simulink model "bldc_current_control"  (R2026a)
settings: Solver=FixedStepDiscrete  StopTime=5  FixedStep=Ts_sim
InitFcn:
  | warning('off','physmod:simscape:engine:core:advancer_errors:fallback_solve')
model workspace (MAT data in the model file):
  B_rotor = 2e-07
  B_turntable = 5e-06
  C_buck = 4.7e-05
  Dmax = 0.95
  Fsw = 50000
  I_max = 1.5
  J_body = 0.002
  J_flywheel = 0.00012
  J_rotor = 5e-07
  K_A = 1
  Ki_current = 7539.82236862
  Ki_speed = 4.0575
  Kp_current = 0.753982236862
  Kp_speed = 0.111675
  L_buck = 0.0001
  T_brk_turntable = 0.0012
  T_col_turntable = 0.001
  Ts_inner = 1e-05
  Ts_outer = 0.01
  Ts_sim = 2e-06
  Vin = 12
  f_pwm = 5000
  psi_m = 0.004
  slew_acc_max = 1.2
  slew_rate_max = 0.5
  w_bias = 0
  w_max = 600
libraries: nesl_utility x18, fl_lib x17, ee_lib x13, slpidlib x3, simulink x1, eePwmGenerator x1
(part 1 of 2)
settings Model: Creator=mulusoy  LastModifiedBy=tama
settings SimscapeCC: SimscapeNominalValues="[{\"value\":\"1\",\"unit\":\"A\"},{\"value\":\"1\",\"unit\":\"bar\"},{\"value\":\"1\",\"unit\":\"cm^2\"},{\"value\":\"1\",\"unit\":\"cm^3/s\"},{\"value\":\"1\",\"unit\":\"kJ/kg\"},{\"value\":\"1\",\"unit\":\"kW\"},{\"value\":\"1\",\"unit\":\"l\"},{\"value\":\"1\",\"unit\":\"N\"},{\"value\":\"1\",\"unit\":\"N*m\"},{\"value\":\"1\",\"unit\":\"V\"}]"  SimscapeLogType=none  SimscapeLogDataHistory=5000.0

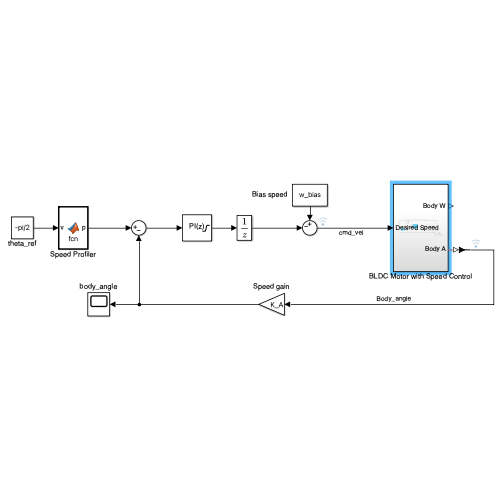
[thumbnail: Simulink's stored preview of the top-level diagram]
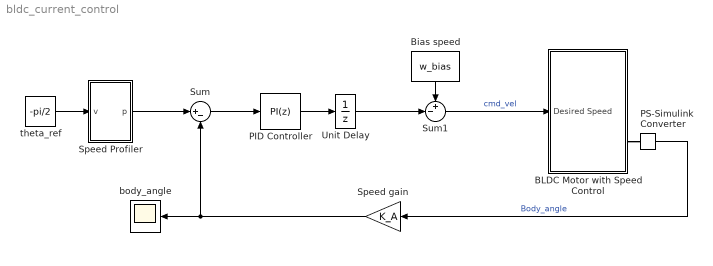
== system bldc_current_control ==
  BLDC Motor with Speed Control : Subsystem
  Bias speed : Constant  Value=w_bias
  PID Controller : slpidlib/PID Controller  Controller=PI  Form=Parallel  TimeDomain=Discrete-time  UseExternalTs=off  SampleTime=0.01  IntegratorMethod=Forward Euler  FilterMethod=Forward Euler  ControllerParametersSource=internal  P=2861  I=6984  UseKiTs=off  D=0  UseExternalDerivativeSource=off  N=100  UseFilter=on  TunerSelectOption=Transfer Function Based (PID Tuner App)  InitialConditionSource=internal  InitialConditionForIntegrator=0  InitialConditionForFilter=0  DifferentiatorICPrevScaledInput=0  ExternalReset=none  TrackingMode=off  Kt=1  LimitOutput=on  SatLimitsSource=internal  UpperSaturationLimit=w_max  LowerSaturationLimit=-w_max  LinearizeAsGain=on  AntiWindupMode=clamping  Kb=1  LimitIntegrator=off  UpperIntegratorSaturationLimit=inf  LowerIntegratorSaturationLimit=-inf  POutMin=[]  POutMax=[]  IOutMin=[]  IOutMax=[]  DOutMin=[]  DOutMax=[]  NOutMin=[]  NOutMax=[]  SumOutMin=[]  SumOutMax=[]  SaturationOutMin=[]  SaturationOutMax=[]  PParamMin=[]  PParamMax=[]  IParamMin=[]  IParamMax=[]  DParamMin=[]  DParamMax=[]  NParamMin=[]  NParamMax=[]  KbParamMin=[]  KbParamMax=[]  KtParamMin=[]  KtParamMax=[]  KbOutMin=[]  KbOutMax=[]  KtOutMin=[]  KtOutMax=[]  IntegratorOutMin=[]  IntegratorOutMax=[]  FilterOutMin=[]  FilterOutMax=[]  SumI1OutMin=[]  SumI1OutMax=[]  SumI2OutMin=[]  SumI2OutMax=[]  SumI3OutMin=[]  SumI3OutMax=[]  SumI4OutMin=[]  SumI4OutMax=[]  SumDOutMin=[]  SumDOutMax=[]  DifferentiatorOutMin=[]  DifferentiatorOutMax=[]  FilterDiffOutCoefMin=[]  FilterDiffOutCoefMax=[]  ReciprocalOutMin=[]  ReciprocalOutMax=[]  SumDenOutMin=[]  SumDenOutMax=[]  SumNumOutMin=[]  SumNumOutMax=[]  DivideOutMin=[]  DivideOutMax=[]  UdiffTsProdOutMin=[]  UdiffTsProdOutMax=[]  NTsProdOutMin=[]  NTsProdOutMax=[]  UintegralTsProdOutMin=[]  UintegralTsProdOutMax=[]  UngainTsProdOutMin=[]  UngainTsProdOutMax=[]  ClampingZeroOutDataTypeStr=Inherit: Inherit via back propagation  ClampingZeroOutMin=[]  ClampingZeroOutMax=[]  FilterDenConstantOutDataTypeStr=Inherit: Inherit via back propagation  FilterDenConstantOutMin=[]  FilterDenConstantOutMax=[]  PCopyOutDataTypeStr=Inherit: Inherit via back propagation  PCopyOutMin=[]  PCopyOutMax=[]  NCopyOutDataTypeStr=Inherit: Inherit via back propagation  NCopyOutMin=[]  NCopyOutMax=[]  IntegratorContinuousStateAttributes=''  IntegratorStateMustResolveToSignalObject=off  IntegratorRTWStateStorageClass=Auto  FilterContinuousStateAttributes=''  FilterStateMustResolveToSignalObject=off  FilterRTWStateStorageClass=Auto  ParallelPVariant=InternalParameters  IdealPVariant=Disabled  IVariant=InternalParameters  DVariant=Disabled  IntegratorVariant=Discrete  SatVariant=Enabled  AWVariant=DiscClampingParallel  PCopyVariant=Disabled  TRVariant=Disabled  FdbkBlocksVariant=Forward  IdealPFdbkVariant=Disabled  SatFdbkVariant=Disabled  DerivativeFilterVariant=Disabled  NVariant=Disabled  NCopyVariant=Disabled_SignalSpec  FilterICVariant=Disabled  IntegratorICVariant=InternalICs  ExternalResetVariant=Disabled  TRSumVariant=Passthrough  SumFdbkVariant=Disabled  SumVariant=Sum_PI  TsampFilterVariant=InternalTs  TsampNgainVariant=Passthrough  TsampIntegralVariant=Disabled_SignalSpec  ExternalSaturationOutDataTypeStr=Inherit: Same as second input  DerivativeSourceVariant=Disabled  PreIntVariant=InternalPreInt
  PS-Simulink Converter : nesl_utility/PS-Simulink Converter  PhysicalDomain=network_engine_domain  SubClassName=ps_output  LeftPortType=input  RightPortType=output  PseudoPeriodic=off  Frequencies=[]  VectorFormat=inherit  Unit=inherit  AffineConversion=off
  Speed Profiler : MATLAB Function  TreatAsAtomicUnit=on  SystemSampleTime=Ts_outer
  Speed gain : Gain  Gain=K_A
  Sum : Sum  Inputs=|+-
  Sum1 : Sum  Inputs=+-|
  Unit Delay : UnitDelay  SampleTime=-1
  body_angle : Scope
      settings: ActiveDisplayYMinimum=-1.3977070447201263  ActiveDisplayYMaximum=0.52158832632188012  DataLoggingVariableName=ScopeData3
  theta_ref : Constant  Value=-pi/2
  wires:
  PID Controller/1 -> Unit Delay/1
  PS-Simulink Converter/1 -> Speed gain/1  "Body_angle"
  theta_ref/1 -> Speed Profiler/1(v)
  Sum/1 -> PID Controller/1
  Speed gain/1 -> Sum/2, body_angle/1
  Bias speed/1 -> Sum1/1
  Unit Delay/1 -> Sum1/2
  Sum1/1 -> BLDC Motor with Speed Control/1(Desired Speed)  "cmd_vel"
  Speed Profiler/1(p) -> Sum/1
  connections:
  BLDC Motor with Speed Control/RConn2 -- PS-Simulink Converter/LConn1

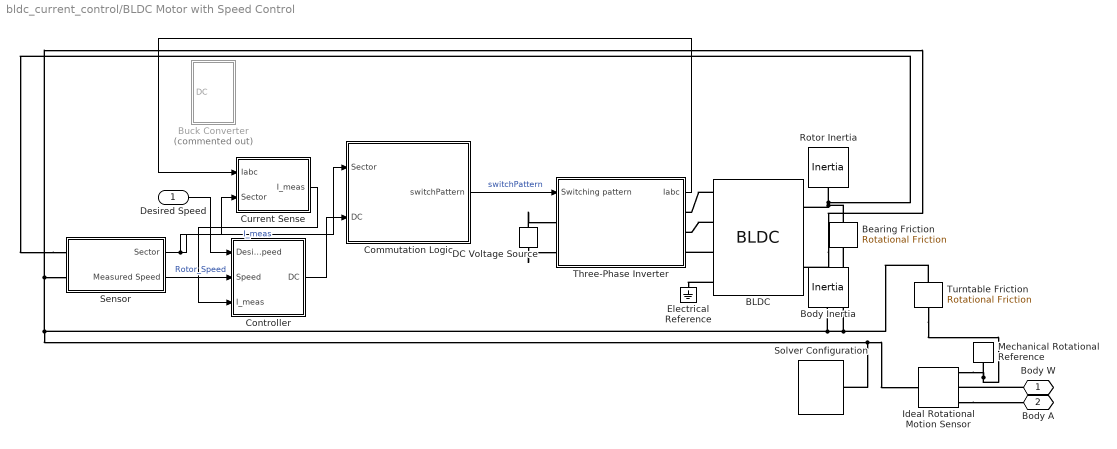
== system bldc_current_control/BLDC Motor with Speed Control ==
  Desired Speed : Inport
  BLDC : ee_lib/Electromechanical/Permanent Magnet/BLDC  port_option=ee.enum.threePhasePort.expanded  rotor_param=1  pm_flux_linkage=psi_m Wb  theta_constant=120/1 deg  emf_max=9.6 V  w_meas=600 rpm  DphiDtheta_tab=[0, -.1528, -.1528, .1528, .1528, 0] Wb/rad  back_emf_tab=[0, -9.6, -9.6, 9.6, 9.6, 0] V  rotor_angle_tab=[0, 7.5, 22.5, 37.5, 52.5, 60] deg  nPolePairs=1  axes_param=2  winding_type=ee.enum.statorconnection.wye  stator_param=ee.enum.statorparam.LdLqL0  machine_param=ee.enum.dqparameterization.constant  Ld=0.2 mH  Lq=0.2 mH  idVec=[-200, 0, 200] A  iqVec=[-200, 0, 200] A  LdMatrix=0.00022 * ones(3, 3) H  LqMatrix=0.00022 * ones(3, 3) H  L0=0.2 mH  Ls=0.0002 H  Lm=0 H  Ms=0.00002 H  Rs=2 Ohm  zero_sequence=ee.enum.park.zerosequence.include  loss_param=ee.enum.ironloss.none  losses_oc=[0, 0, 0] W  losses_sc=[0, 0, 0] W  f_losses=60 Hz  Isc_losses=95 A  J=0 kg*m^2  lam=B_rotor N*m/(rad/s)  i_d_specify=off  i_d_priority=None  i_d=0 A  i_d_nominal_specify=off  i_d_nominal_value=1  i_d_nominal_unit=A  i_q_specify=off  i_q_priority=None  i_q=0 A  i_q_nominal_specify=off  i_q_nominal_value=1  i_q_nominal_unit=A  torque_specify=off  torque_priority=None  torque=0 N*m  torque_nominal_specify=off  torque_nominal_value=1  torque_nominal_unit=N*m  angular_velocity_specify=on  angular_velocity_priority=High  angular_velocity=w_bias rpm  angular_velocity_nominal_specify=off  angular_velocity_nominal_value=1  angular_velocity_nominal_unit=rpm  angular_position_specify=off  angular_position_priority=High  angular_position=0 deg  angular_position_nominal_specify=off  angular_position_nominal_value=1  angular_position_nominal_unit=deg  alpha=3.93e-3 1/K  alpha_flux=-0.001 1/K  Tmeas=298.15 K  stator_thermal_mass=100 J/K  rotor_thermal_mass=200 J/K  Rm_percent_rotor=90  Rd_percent_rotor=30  temperatureA_specify=off  temperatureA_priority=High  temperatureA=25 degC  temperatureA_nominal_specify=off  temperatureA_nominal_value=1  temperatureA_nominal_unit=degC  temperatureB_specify=off  temperatureB_priority=High  temperatureB=25 degC  temperatureB_nominal_specify=off  temperatureB_nominal_value=1  temperatureB_nominal_unit=degC  temperatureC_specify=off  temperatureC_priority=High  temperatureC=25 degC  temperatureC_nominal_specify=off  temperatureC_nominal_value=1  temperatureC_nominal_unit=degC  temperatureR_specify=off  temperatureR_priority=High  temperatureR=25 degC  temperatureR_nominal_specify=off  temperatureR_nominal_value=1  temperatureR_nominal_unit=degC
  Bearing Friction : fl_lib/Mechanical/Rotational Elements/Rotational Friction  brkwy_trq=0.05 m*mN  brkwy_vel=0.1 rad/s  Col_trq=0.05 m*mN  visc_coef=0 N*m*s/rad  w_specify=off  w_priority=None  w=0 rad/s  w_nominal_specify=off  w_nominal_value=1  w_nominal_unit=rad/s  t_specify=off  t_priority=None  t=0 N*m  t_nominal_specify=off  t_nominal_value=1  t_nominal_unit=N*m
  Body Inertia : fl_lib/Mechanical/Rotational Elements/Inertia  inertia=J_body kg*m^2  num_ports=foundation.enum.numPorts2.one  w_specify=on  w_priority=High  w=0 rad/s  w_nominal_specify=off  w_nominal_value=1  w_nominal_unit=rad/s  t_specify=off  t_priority=None  t=0 N*m  t_nominal_specify=off  t_nominal_value=1  t_nominal_unit=N*m
  Buck Converter : Subsystem  Description=Label-mode variant. Averaged (default): Vin*d controlled source + L/C filter, run with Ts_sim = 1e-5. Switching: PWM + MOSFETs at Fsw, needs Ts_sim <= 2e-7 (1% duty resolution at 50 kHz) - set Ts_sim in the model workspace before switching.  Commented=on  Variant=on  VariantControlMode=label  LabelModeActiveChoice=Averaged
  Commutation Logic : Subsystem
  Controller : Subsystem
  Current Sense : Subsystem
  DC Voltage Source : ee_lib/Additional Components/SPICE Sources/DC Voltage Source  DC=Vin V
  Electrical Reference : fl_lib/Electrical/Electrical Elements/Electrical Reference
  Ideal Rotational Motion Sensor : fl_lib/Mechanical/Mechanical Sensors/Ideal Rotational Motion Sensor  reference=foundation.enum.MeasurementReference.difference  acceleration_port=false  velocity_port=true  position_port=true  wrap_angle=false  offset=0 rad
  Mechanical Rotational Reference : fl_lib/Mechanical/Rotational Elements/Mechanical Rotational Reference
  Rotor Inertia : fl_lib/Mechanical/Rotational Elements/Inertia  inertia=J_flywheel + J_rotor kg*m^2  num_ports=foundation.enum.numPorts2.one  w_specify=on  w_priority=High  w=w_bias rpm  w_nominal_specify=off  w_nominal_value=1  w_nominal_unit=rad/s  t_specify=off  t_priority=None  t=0 N*m  t_nominal_specify=off  t_nominal_value=1  t_nominal_unit=N*m
  Sensor : Subsystem
  Solver Configuration : nesl_utility/Solver Configuration  PhysicalDomain=network_engine_domain  SubClassName=solver  LeftPortType=input  RightPortType=generic  Tones=[]  Harmonics=[]  SimulateNoise=off  Profile=off  UseLocalSampling=off  EnableSwitchedLinearOptims=on  FrequencyDomain=off  UseCCode=off  RelTol=0.001  AbsTol=1e-06  MinStep=1e-09  ToWorkspace=off  RevertToSquareIcSolve=off  NumHomotopyIterations=100  PhasorMode=off  PhasorModeNumHarmonics=1  ConsistencySolver=NEWTON_FTOL  CanonicalOrdering=UNORDERED  OptimizeIntermediates=UNOPTIMIZED  IndexReductionMethod=DerivativeReplacement  DoDC=off  ResidualTolerance=1e-09  ConsistencyTolSource=GLOBAL  ConsistencyAbsTol=0.001  ConsistencyRelTol=0.001  ConsistencyTolFactor=0.001  UseLocalSolver=on  LocalSolverChoice=NE_BACKWARD_EULER_ADVANCER  ResolveIndetEquations=on  FunctionEvalNumThread=1  LocalSolverSampleTime=Ts_sim  DoFixedCost=on  MaxNonlinIter=4  MaxModeIter=2  ComputeImpulses=off  ImpulseIterations=2  LinearAlgebra=auto  LinearAlgebraNumThread=0  EquationFormulation=NE_TIME_EF  DelaysMemoryBudget=1024  AutomaticFiltering=off  FilteringTimeConstant=0.001  PartitionStorageMethod=AS_NEEDED  PartitionMemoryBudget=1024  PartitionMethod=ROBUST  MultibodyUseLocalSolver=off  MultibodyLocalSolverChoice=ODE1  MultibodyLocalSolverSampleTime=0.001
  Three-Phase Inverter : Subsystem
  Turntable Friction : fl_lib/Mechanical/Rotational Elements/Rotational Friction  brkwy_trq=T_brk_turntable N*m  brkwy_vel=0.1 rad/s  Col_trq=T_col_turntable N*m  visc_coef=B_turntable N*m*s/rad  w_specify=off  w_priority=None  w=0 rad/s  w_nominal_specify=off  w_nominal_value=1  w_nominal_unit=rad/s  t_specify=off  t_priority=None  t=0 N*m  t_nominal_specify=off  t_nominal_value=1  t_nominal_unit=N*m
  Body W : PMIOPort  Side=Right
  Body A : PMIOPort  Port=2  Side=Right
  wires:
  Commutation Logic/1(switchPattern) -> Three-Phase Inverter/1(Switching pattern)  "switchPattern"
  Current Sense/1(I_meas) -> Controller/3(I_meas)  "I_meas"
  Three-Phase Inverter/1(Iabc) -> Current Sense/1(Iabc)
  Desired Speed/1 -> Controller/1(Desired Speed)
  Controller/1(DC) -> Commutation Logic/2(DC)
  Sensor/1(Sector) -> Current Sense/2(Sector), Commutation Logic/1(Sector)
  Sensor/2(Measured Speed) -> Controller/2(Speed)  "Rotor_Speed"
  connections:
  BLDC/LConn2 -- Three-Phase Inverter/RConn2
  BLDC/LConn1 -- Three-Phase Inverter/RConn1
  BLDC/LConn4 -- Electrical Reference/LConn1
  BLDC/LConn3 -- Three-Phase Inverter/RConn3
  Mechanical Rotational Reference/LConn1 -- Ideal Rotational Motion Sensor/RConn1 -- Turntable Friction/RConn1
  Body W/RConn1 -- Ideal Rotational Motion Sensor/RConn2
  Ideal Rotational Motion Sensor/RConn3 -- Body A/RConn1
  DC Voltage Source/LConn1 -- Three-Phase Inverter/LConn1
  DC Voltage Source/RConn1 -- Three-Phase Inverter/LConn2
  Sensor/LConn1 -- Bearing Friction/LConn1 -- BLDC/RConn1 -- Rotor Inertia/LConn1
  Body Inertia/LConn1 -- Ideal Rotational Motion Sensor/LConn1 -- Solver Configuration/RConn1 -- Turntable Friction/LConn1 -- Bearing Friction/RConn1 -- BLDC/RConn2 -- Sensor/LConn2

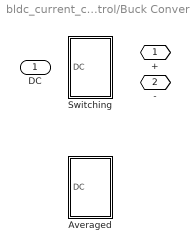
== system bldc_current_control/BLDC Motor with Speed Control/Buck Converter ==
  DC : Inport
  Averaged : Subsystem  VariantControl=Averaged
  Switching : Subsystem  VariantControl=Switching
  + : PMIOPort  Side=Right
  - : PMIOPort  Port=2  Side=Right

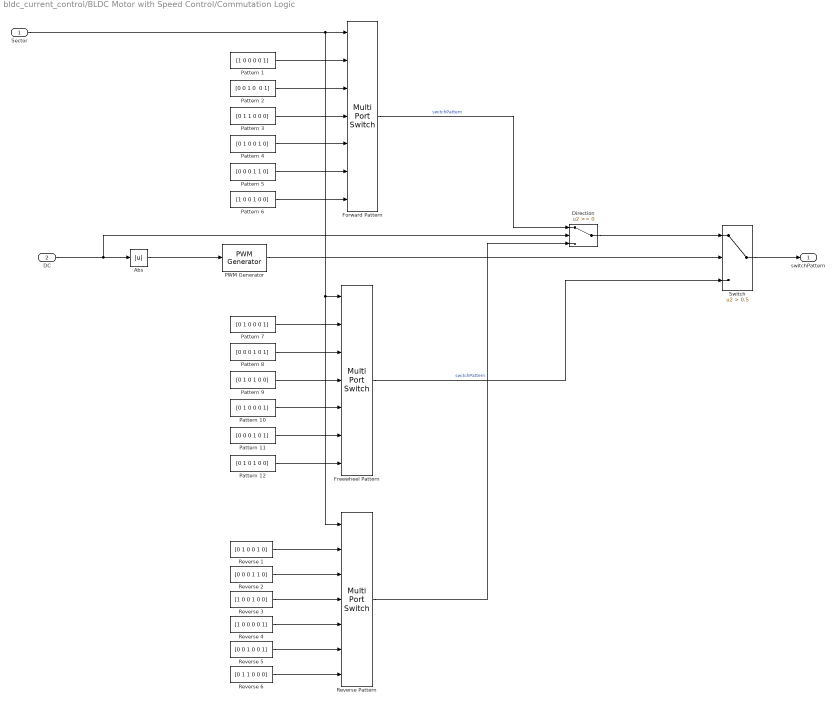
== system bldc_current_control/BLDC Motor with Speed Control/Commutation Logic ==
  Sector : Inport
  DC : Inport  Port=2
  Abs : Abs  SaturateOnIntegerOverflow=off
  Direction : Switch  SaturateOnIntegerOverflow=off  InputSameDT=off
  Forward Pattern : MultiPortSwitch  Inputs=6  SaturateOnIntegerOverflow=off  InputSameDT=off
  Freewheel Pattern : MultiPortSwitch  Inputs=6  SaturateOnIntegerOverflow=off  InputSameDT=off
  PWM Generator : eePwmGenerator/PWM Generator  CarrCount=Up  Tper=1/f_pwm  Tdelay=0  Ts=Ts_sim
  Pattern 1 : Constant  Value=[1 0 0 0 0 1]
  Pattern 10 : Constant  Value=[0 1 0 0 0 1]
  Pattern 11 : Constant  Value=[0 0 0 1 0 1]
  Pattern 12 : Constant  Value=[0 1 0 1 0 0]
  Pattern 2 : Constant  Value="[0 0 1 0  0 1]"
  Pattern 3 : Constant  Value=[0 1 1 0 0 0]
  Pattern 4 : Constant  Value=[0 1 0 0 1 0]
  Pattern 5 : Constant  Value=[0 0 0 1 1 0]
  Pattern 6 : Constant  Value=[1 0 0 1 0 0]
  Pattern 7 : Constant  Value=[0 1 0 0 0 1]
  Pattern 8 : Constant  Value=[0 0 0 1 0 1]
  Pattern 9 : Constant  Value=[0 1 0 1 0 0]
  Reverse 1 : Constant  Value=[0 1 0 0 1 0]
  Reverse 2 : Constant  Value=[0 0 0 1 1 0]
  Reverse 3 : Constant  Value=[1 0 0 1 0 0]
  Reverse 4 : Constant  Value=[1 0 0 0 0 1]
  Reverse 5 : Constant  Value=[0 0 1 0 0 1]
  Reverse 6 : Constant  Value=[0 1 1 0 0 0]
  Reverse Pattern : MultiPortSwitch  Inputs=6  SaturateOnIntegerOverflow=off  InputSameDT=off
  Switch : Switch  Criteria=u2 > Threshold  Threshold=0.5  SaturateOnIntegerOverflow=off  InputSameDT=off
  switchPattern : Outport
  wires:
  Pattern 12/1 -> Freewheel Pattern/7
  Pattern 10/1 -> Freewheel Pattern/5
  Pattern 8/1 -> Freewheel Pattern/3
  Pattern 11/1 -> Freewheel Pattern/6
  Pattern 9/1 -> Freewheel Pattern/4
  Freewheel Pattern/1 -> Switch/3  "switchPattern"
  Switch/1 -> switchPattern/1
  Abs/1 -> PWM Generator/1
  Direction/1 -> Switch/1
  Reverse Pattern/1 -> Direction/3
  Reverse 6/1 -> Reverse Pattern/7
  Reverse 5/1 -> Reverse Pattern/6
  Reverse 4/1 -> Reverse Pattern/5
  Reverse 3/1 -> Reverse Pattern/4
  Reverse 2/1 -> Reverse Pattern/3
  Reverse 1/1 -> Reverse Pattern/2
  PWM Generator/1 -> Switch/2
  DC/1 -> Direction/2, Abs/1
  Pattern 7/1 -> Freewheel Pattern/2
  Sector/1 -> Forward Pattern/1, Freewheel Pattern/1, Reverse Pattern/1
  Pattern 1/1 -> Forward Pattern/2
  Pattern 6/1 -> Forward Pattern/7
  Forward Pattern/1 -> Direction/1  "switchPattern"
  Pattern 4/1 -> Forward Pattern/5
  Pattern 2/1 -> Forward Pattern/3
  Pattern 5/1 -> Forward Pattern/6
  Pattern 3/1 -> Forward Pattern/4

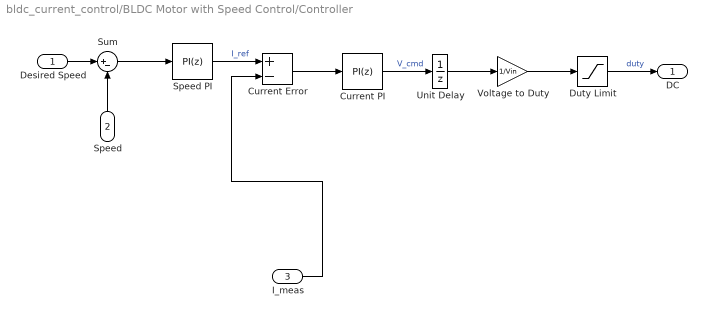
== system bldc_current_control/BLDC Motor with Speed Control/Controller ==
  Desired Speed : Inport
  Speed : Inport  Port=2
  I_meas : Inport  Port=3
  Current Error : Sum  Inputs=+-
  Current PI : slpidlib/PID Controller  Controller=PI  Form=Parallel  TimeDomain=Discrete-time  UseExternalTs=off  SampleTime=Ts_inner  IntegratorMethod=Forward Euler  FilterMethod=Forward Euler  ControllerParametersSource=internal  P=Kp_current  I=Ki_current  UseKiTs=off  D=0  UseExternalDerivativeSource=off  N=100  UseFilter=on  TunerSelectOption=Transfer Function Based (PID Tuner App)  InitialConditionSource=internal  InitialConditionForIntegrator=0  InitialConditionForFilter=0  DifferentiatorICPrevScaledInput=0  ExternalReset=none  TrackingMode=off  Kt=1  LimitOutput=on  SatLimitsSource=internal  UpperSaturationLimit=Dmax*Vin  LowerSaturationLimit=-Dmax*Vin  LinearizeAsGain=on  AntiWindupMode=clamping  Kb=1  LimitIntegrator=off  UpperIntegratorSaturationLimit=inf  LowerIntegratorSaturationLimit=-inf  POutMin=[]  POutMax=[]  IOutMin=[]  IOutMax=[]  DOutMin=[]  DOutMax=[]  NOutMin=[]  NOutMax=[]  SumOutMin=[]  SumOutMax=[]  SaturationOutMin=[]  SaturationOutMax=[]  PParamMin=[]  PParamMax=[]  IParamMin=[]  IParamMax=[]  DParamMin=[]  DParamMax=[]  NParamMin=[]  NParamMax=[]  KbParamMin=[]  KbParamMax=[]  KtParamMin=[]  KtParamMax=[]  KbOutMin=[]  KbOutMax=[]  KtOutMin=[]  KtOutMax=[]  IntegratorOutMin=[]  IntegratorOutMax=[]  FilterOutMin=[]  FilterOutMax=[]  SumI1OutMin=[]  SumI1OutMax=[]  SumI2OutMin=[]  SumI2OutMax=[]  SumI3OutMin=[]  SumI3OutMax=[]  SumI4OutMin=[]  SumI4OutMax=[]  SumDOutMin=[]  SumDOutMax=[]  DifferentiatorOutMin=[]  DifferentiatorOutMax=[]  FilterDiffOutCoefMin=[]  FilterDiffOutCoefMax=[]  ReciprocalOutMin=[]  ReciprocalOutMax=[]  SumDenOutMin=[]  SumDenOutMax=[]  SumNumOutMin=[]  SumNumOutMax=[]  DivideOutMin=[]  DivideOutMax=[]  UdiffTsProdOutMin=[]  UdiffTsProdOutMax=[]  NTsProdOutMin=[]  NTsProdOutMax=[]  UintegralTsProdOutMin=[]  UintegralTsProdOutMax=[]  UngainTsProdOutMin=[]  UngainTsProdOutMax=[]  ClampingZeroOutDataTypeStr=Inherit: Inherit via back propagation  ClampingZeroOutMin=[]  ClampingZeroOutMax=[]  FilterDenConstantOutDataTypeStr=Inherit: Inherit via back propagation  FilterDenConstantOutMin=[]  FilterDenConstantOutMax=[]  PCopyOutDataTypeStr=Inherit: Inherit via back propagation  PCopyOutMin=[]  PCopyOutMax=[]  NCopyOutDataTypeStr=Inherit: Inherit via back propagation  NCopyOutMin=[]  NCopyOutMax=[]  IntegratorContinuousStateAttributes=''  IntegratorStateMustResolveToSignalObject=off  IntegratorRTWStateStorageClass=Auto  FilterContinuousStateAttributes=''  FilterStateMustResolveToSignalObject=off  FilterRTWStateStorageClass=Auto  ParallelPVariant=InternalParameters  IdealPVariant=Disabled  IVariant=InternalParameters  DVariant=Disabled  IntegratorVariant=Discrete  SatVariant=Enabled  AWVariant=DiscClampingParallel  PCopyVariant=Disabled  TRVariant=Disabled  FdbkBlocksVariant=Forward  IdealPFdbkVariant=Disabled  SatFdbkVariant=Disabled  DerivativeFilterVariant=Disabled  NVariant=Disabled  NCopyVariant=Disabled_SignalSpec  FilterICVariant=Disabled  IntegratorICVariant=InternalICs  ExternalResetVariant=Disabled  TRSumVariant=Passthrough  SumFdbkVariant=Disabled  SumVariant=Sum_PI  TsampFilterVariant=InternalTs  TsampNgainVariant=Passthrough  TsampIntegralVariant=Disabled_SignalSpec  ExternalSaturationOutDataTypeStr=Inherit: Same as second input  DerivativeSourceVariant=Disabled  PreIntVariant=InternalPreInt
  Duty Limit : Saturate  UpperLimit=Dmax  LowerLimit=-Dmax
  Speed PI : slpidlib/PID Controller  Controller=PI  Form=Parallel  TimeDomain=Discrete-time  UseExternalTs=off  SampleTime=Ts_inner  IntegratorMethod=Forward Euler  FilterMethod=Forward Euler  ControllerParametersSource=internal  P=Kp_speed  I=Ki_speed  UseKiTs=off  D=0  UseExternalDerivativeSource=off  N=100  UseFilter=on  TunerSelectOption=Transfer Function Based (PID Tuner App)  InitialConditionSource=internal  InitialConditionForIntegrator=0  InitialConditionForFilter=0  DifferentiatorICPrevScaledInput=0  ExternalReset=none  TrackingMode=off  Kt=1  LimitOutput=on  SatLimitsSource=internal  UpperSaturationLimit=I_max  LowerSaturationLimit=-I_max  LinearizeAsGain=on  AntiWindupMode=clamping  Kb=1  LimitIntegrator=off  UpperIntegratorSaturationLimit=inf  LowerIntegratorSaturationLimit=-inf  POutMin=[]  POutMax=[]  IOutMin=[]  IOutMax=[]  DOutMin=[]  DOutMax=[]  NOutMin=[]  NOutMax=[]  SumOutMin=[]  SumOutMax=[]  SaturationOutMin=[]  SaturationOutMax=[]  PParamMin=[]  PParamMax=[]  IParamMin=[]  IParamMax=[]  DParamMin=[]  DParamMax=[]  NParamMin=[]  NParamMax=[]  KbParamMin=[]  KbParamMax=[]  KtParamMin=[]  KtParamMax=[]  KbOutMin=[]  KbOutMax=[]  KtOutMin=[]  KtOutMax=[]  IntegratorOutMin=[]  IntegratorOutMax=[]  FilterOutMin=[]  FilterOutMax=[]  SumI1OutMin=[]  SumI1OutMax=[]  SumI2OutMin=[]  SumI2OutMax=[]  SumI3OutMin=[]  SumI3OutMax=[]  SumI4OutMin=[]  SumI4OutMax=[]  SumDOutMin=[]  SumDOutMax=[]  DifferentiatorOutMin=[]  DifferentiatorOutMax=[]  FilterDiffOutCoefMin=[]  FilterDiffOutCoefMax=[]  ReciprocalOutMin=[]  ReciprocalOutMax=[]  SumDenOutMin=[]  SumDenOutMax=[]  SumNumOutMin=[]  SumNumOutMax=[]  DivideOutMin=[]  DivideOutMax=[]  UdiffTsProdOutMin=[]  UdiffTsProdOutMax=[]  NTsProdOutMin=[]  NTsProdOutMax=[]  UintegralTsProdOutMin=[]  UintegralTsProdOutMax=[]  UngainTsProdOutMin=[]  UngainTsProdOutMax=[]  ClampingZeroOutDataTypeStr=Inherit: Inherit via back propagation  ClampingZeroOutMin=[]  ClampingZeroOutMax=[]  FilterDenConstantOutDataTypeStr=Inherit: Inherit via back propagation  FilterDenConstantOutMin=[]  FilterDenConstantOutMax=[]  PCopyOutDataTypeStr=Inherit: Inherit via back propagation  PCopyOutMin=[]  PCopyOutMax=[]  NCopyOutDataTypeStr=Inherit: Inherit via back propagation  NCopyOutMin=[]  NCopyOutMax=[]  IntegratorContinuousStateAttributes=''  IntegratorStateMustResolveToSignalObject=off  IntegratorRTWStateStorageClass=Auto  FilterContinuousStateAttributes=''  FilterStateMustResolveToSignalObject=off  FilterRTWStateStorageClass=Auto  ParallelPVariant=InternalParameters  IdealPVariant=Disabled  IVariant=InternalParameters  DVariant=Disabled  IntegratorVariant=Discrete  SatVariant=Enabled  AWVariant=DiscClampingParallel  PCopyVariant=Disabled  TRVariant=Disabled  FdbkBlocksVariant=Forward  IdealPFdbkVariant=Disabled  SatFdbkVariant=Disabled  DerivativeFilterVariant=Disabled  NVariant=Disabled  NCopyVariant=Disabled_SignalSpec  FilterICVariant=Disabled  IntegratorICVariant=InternalICs  ExternalResetVariant=Disabled  TRSumVariant=Passthrough  SumFdbkVariant=Disabled  SumVariant=Sum_PI  TsampFilterVariant=InternalTs  TsampNgainVariant=Passthrough  TsampIntegralVariant=Disabled_SignalSpec  ExternalSaturationOutDataTypeStr=Inherit: Same as second input  DerivativeSourceVariant=Disabled  PreIntVariant=InternalPreInt
  Sum : Sum  Inputs=|+-
  Unit Delay : UnitDelay  SampleTime=-1
  Voltage to Duty : Gain  Gain=1/Vin
  DC : Outport
  wires:
  Speed/1 -> Sum/2
  Desired Speed/1 -> Sum/1
  Current PI/1 -> Unit Delay/1  "V_cmd"
  Current Error/1 -> Current PI/1
  I_meas/1 -> Current Error/2
  Speed PI/1 -> Current Error/1  "I_ref"
  Voltage to Duty/1 -> Duty Limit/1
  Sum/1 -> Speed PI/1
  Unit Delay/1 -> Voltage to Duty/1
  Duty Limit/1 -> DC/1  "duty"

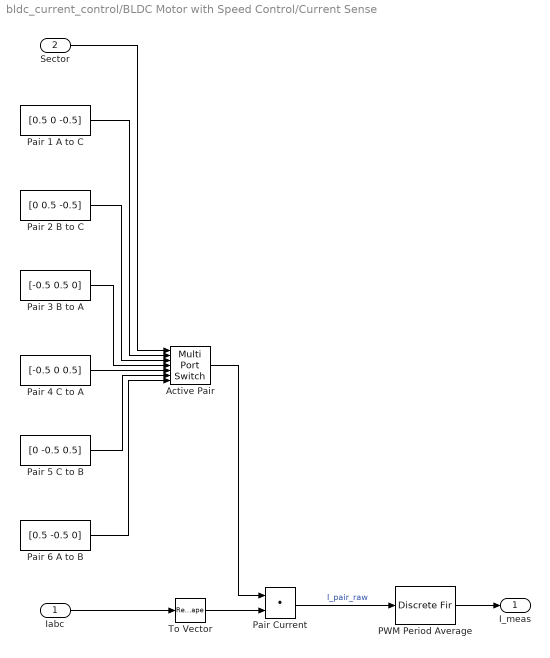
== system bldc_current_control/BLDC Motor with Speed Control/Current Sense ==
  Iabc : Inport
  Sector : Inport  Port=2
  Active Pair : MultiPortSwitch  Inputs=6  SaturateOnIntegerOverflow=off  InputSameDT=off
  PWM Period Average : DiscreteFir  Coefficients=ones(1,round(1/(f_pwm*Ts_sim)))/round(1/(f_pwm*Ts_sim))
  Pair 1 A to C : Constant  Value=[0.5 0 -0.5]
  Pair 2 B to C : Constant  Value=[0 0.5 -0.5]
  Pair 3 B to A : Constant  Value=[-0.5 0.5 0]
  Pair 4 C to A : Constant  Value=[-0.5 0 0.5]
  Pair 5 C to B : Constant  Value=[0 -0.5 0.5]
  Pair 6 A to B : Constant  Value=[0.5 -0.5 0]
  Pair Current : DotProduct  OutDataTypeStr=Inherit: Inherit via internal rule
  To Vector : Reshape
  I_meas : Outport
  wires:
  PWM Period Average/1 -> I_meas/1
  Pair Current/1 -> PWM Period Average/1  "I_pair_raw"
  To Vector/1 -> Pair Current/2
  Active Pair/1 -> Pair Current/1
  Pair 6 A to B/1 -> Active Pair/7
  Pair 5 C to B/1 -> Active Pair/6
  Pair 4 C to A/1 -> Active Pair/5
  Pair 3 B to A/1 -> Active Pair/4
  Pair 2 B to C/1 -> Active Pair/3
  Pair 1 A to C/1 -> Active Pair/2
  Sector/1 -> Active Pair/1
  Iabc/1 -> To Vector/1

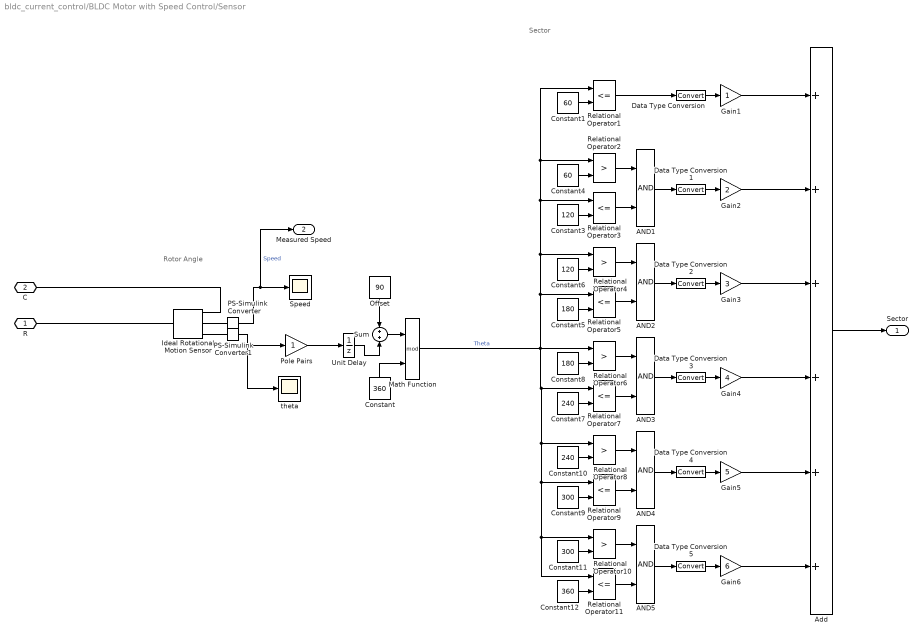
== system bldc_current_control/BLDC Motor with Speed Control/Sensor ==
  note: Rotor Angle
  note: Sector
  AND{1..5} (5 alike) : Logic  AllPortsSameDT=off  OutDataTypeStr=boolean
  Add : Sum  Inputs=6
  Constant : Constant  Value=360
  Constant1 : Constant  Value=60
  Constant10 : Constant  Value=240
  Constant11 : Constant  Value=300
  Constant12 : Constant  Value=360
  Constant3 : Constant  Value=120
  Constant4 : Constant  Value=60
  Constant5 : Constant  Value=180
  Constant6 : Constant  Value=120
  Constant7 : Constant  Value=240
  Constant8 : Constant  Value=180
  Constant9 : Constant  Value=300
  Data Type Conversion{,1..5} (6 alike) : DataTypeConversion  SaturateOnIntegerOverflow=off  RndMeth=Floor
  Gain1 : Gain
  Gain2 : Gain  Gain=2
  Gain3 : Gain  Gain=3
  Gain4 : Gain  Gain=4
  Gain5 : Gain  Gain=5
  Gain6 : Gain  Gain=6
  Ideal Rotational Motion Sensor : fl_lib/Mechanical/Mechanical Sensors/Ideal Rotational Motion Sensor  reference=foundation.enum.MeasurementReference.difference  acceleration_port=false  velocity_port=true  position_port=true  wrap_angle=false  offset=0 deg
  Math Function : Math  Operator=mod
  Offset : Constant  Value=90
  PS-Simulink Converter : nesl_utility/PS-Simulink Converter  PhysicalDomain=network_engine_domain  SubClassName=ps_output  LeftPortType=input  RightPortType=output  PseudoPeriodic=off  Frequencies=[]  VectorFormat=1-D array  Unit=rpm  AffineConversion=off
  PS-Simulink Converter1 : nesl_utility/PS-Simulink Converter  PhysicalDomain=network_engine_domain  SubClassName=ps_output  LeftPortType=input  RightPortType=output  PseudoPeriodic=off  Frequencies=[]  VectorFormat=1-D array  Unit=deg  AffineConversion=off
  Pole Pairs : Gain
  Relational Operator{1,3,5,7,9,11} (6 alike) : RelationalOperator  Operator=<=  OutDataTypeStr=boolean  RndMeth=Simplest  InputSameDT=off
  Relational Operator{2,4,6,8,10} (5 alike) : RelationalOperator  Operator=>  OutDataTypeStr=boolean  RndMeth=Simplest  InputSameDT=off
  Speed : Scope
      settings: ActiveDisplayYMinimum=-51.95479  ActiveDisplayYMaximum=223.68655  DataLoggingVariableName=theta
  Sum : Sum  Inputs=+|+
  Unit Delay : UnitDelay  SampleTime=-1
  theta : Scope
      settings: ActiveDisplayYMinimum=-1  ActiveDisplayYMaximum=1  DataLoggingVariableName=ScopeData2
  R : PMIOPort  Side=Left
  C : PMIOPort  Port=2  Side=Left
  Sector : Outport
  Measured Speed : Outport  Port=2
  wires:
  Add/1 -> Sector/1
  Gain6/1 -> Add/6
  Gain5/1 -> Add/5
  Gain4/1 -> Add/4
  Gain3/1 -> Add/3
  Gain2/1 -> Add/2
  Gain1/1 -> Add/1
  Relational Operator5/1 -> AND2/2
  Relational Operator10/1 -> AND5/1
  AND1/1 -> Data Type Conversion1/1
  Constant11/1 -> Relational Operator10/2
  AND5/1 -> Data Type Conversion5/1
  Constant12/1 -> Relational Operator11/2
  Data Type Conversion/1 -> Gain1/1
  AND2/1 -> Data Type Conversion2/1
  Relational Operator1/1 -> Data Type Conversion/1
  Data Type Conversion2/1 -> Gain3/1
  Data Type Conversion1/1 -> Gain2/1
  Data Type Conversion5/1 -> Gain6/1
  AND3/1 -> Data Type Conversion3/1
  Constant8/1 -> Relational Operator6/2
  Constant7/1 -> Relational Operator7/2
  Relational Operator6/1 -> AND3/1
  Data Type Conversion4/1 -> Gain5/1
  Relational Operator2/1 -> AND1/1
  AND4/1 -> Data Type Conversion4/1
  Relational Operator9/1 -> AND4/2
  Constant5/1 -> Relational Operator5/2
  Relational Operator3/1 -> AND1/2
  Constant3/1 -> Relational Operator3/2
  Relational Operator7/1 -> AND3/2
  Relational Operator4/1 -> AND2/1
  Constant4/1 -> Relational Operator2/2
  Constant1/1 -> Relational Operator1/2
  Data Type Conversion3/1 -> Gain4/1
  Relational Operator8/1 -> AND4/1
  Constant10/1 -> Relational Operator8/2
  Constant6/1 -> Relational Operator4/2
  Constant9/1 -> Relational Operator9/2
  Relational Operator11/1 -> AND5/2
  Math Function/1 -> Relational Operator6/1, Relational Operator1/1, Relational Operator2/1, Relational Operator3/1, Relational Operator4/1, Relational Operator5/1, Relational Operator7/1, Relational Operator8/1, Relational Operator10/1, Relational Operator11/1, Relational Operator9/1  "Theta"
  Pole Pairs/1 -> Unit Delay/1
  PS-Simulink Converter1/1 -> theta/1, Pole Pairs/1
  PS-Simulink Converter/1 -> Measured Speed/1, Speed/1  "Speed"
  Constant/1 -> Math Function/2
  Unit Delay/1 -> Sum/2
  Offset/1 -> Sum/1
  Sum/1 -> Math Function/1
  connections:
  Ideal Rotational Motion Sensor/LConn1 -- R/RConn1
  PS-Simulink Converter/LConn1 -- Ideal Rotational Motion Sensor/RConn2
  Ideal Rotational Motion Sensor/RConn1 -- C/RConn1
  Ideal Rotational Motion Sensor/RConn3 -- PS-Simulink Converter1/LConn1
